simulink model "DCMotor"  (R2024b)
settings: Solver=VariableStepAuto  StartTime=0.0  StopTime=0.2  RelTol=1e-3
values from neighbouring files (symbols this model uses):
  b = 0    [C01A_Parameters.m]    (also in param.m = 0.000180072449898)
  Cn = 0.22    [C01A_Parameters.m]    (also in param.m = 0)
  J = 0.352e-4    (= 3.52e-05)    [C01A_Parameters.m]    (also in param.m)
  Km = 0.11    [C01A_Parameters.m]    (also in param.m)
  L = 4.1e-3    (= 0.0041)    [C01A_Parameters.m]    (also in param.m)
  R = 3.2    [C01A_Parameters.m]    (also in param.m)
  RadToRpm = 60/(2*pi)    (= 9.54929658551)    [C01A_Parameters.m]    (also in param.m)
settings Model: Creator=student  LastModifiedBy=student

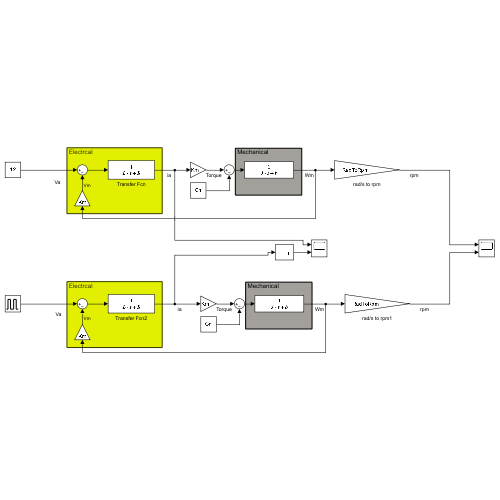
[thumbnail: Simulink's stored preview of the top-level diagram]
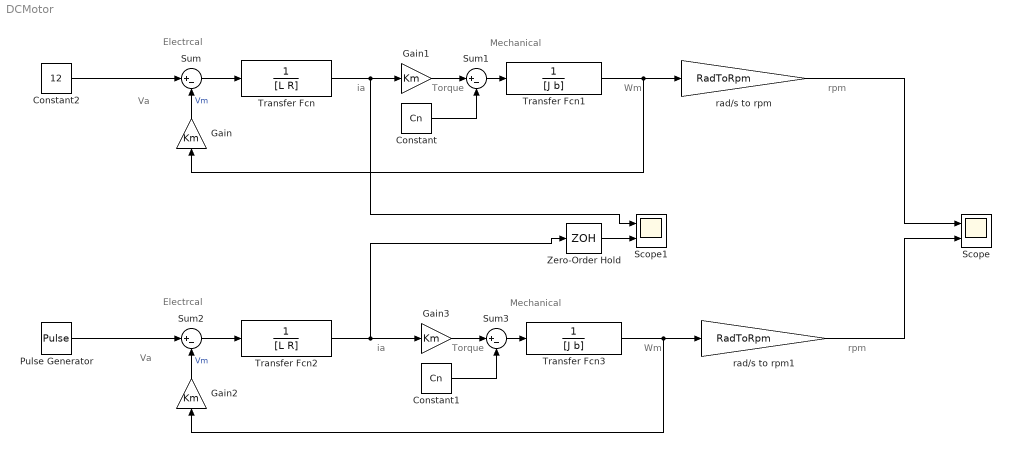
== system DCMotor ==
  note: Mechanical
  note: Electrcal
  note: Va
  note: Torque
  note: ia
  note: Wm
  note: rpm
  note: Wm
  note: Torque
  note: Electrcal
  note: Mechanical
  note: Va
  note: ia
  note: rpm
  Constant : Constant  Value=Cn
  Constant1 : Constant  Value=Cn
  Constant2 : Constant  Value=12
  Gain{,1..3} (4 alike) : Gain  Gain=Km
  Pulse Generator : DiscretePulseGenerator  PulseType=Time based  Amplitude=24  Period=0.001  PulseWidth=50
  Scope : Scope  NumInputPorts=2
  Scope1 : Scope  NumInputPorts=2
  Sum{,1..3} (4 alike) : Sum  Inputs=|+-
  Transfer Fcn : TransferFcn  Denominator=[L R]
  Transfer Fcn1 : TransferFcn  Denominator=[J b]
  Transfer Fcn2 : TransferFcn  Denominator=[L R]
  Transfer Fcn3 : TransferFcn  Denominator=[J b]
  Zero-Order Hold : ZeroOrderHold  SampleTime=-1
  rad/s to rpm : Gain  Gain=RadToRpm
  rad/s to rpm1 : Gain  Gain=RadToRpm
  wires:
  Constant2/1 -> Sum/1
  Gain/1 -> Sum/2  "Vm"
  Sum/1 -> Transfer Fcn/1
  Transfer Fcn/1 -> Scope1/1, Gain1/1
  Transfer Fcn1/1 -> Gain/1, rad/s to rpm/1
  Gain1/1 -> Sum1/1
  rad/s to rpm/1 -> Scope/1
  Sum1/1 -> Transfer Fcn1/1
  Constant/1 -> Sum1/2
  Constant1/1 -> Sum3/2
  Sum3/1 -> Transfer Fcn3/1
  Transfer Fcn3/1 -> Gain2/1, rad/s to rpm1/1
  Sum2/1 -> Transfer Fcn2/1
  Pulse Generator/1 -> Sum2/1
  Transfer Fcn2/1 -> Gain3/1, Zero-Order Hold/1
  Gain3/1 -> Sum3/1
  rad/s to rpm1/1 -> Scope/2
  Gain2/1 -> Sum2/2  "Vm"
  Zero-Order Hold/1 -> Scope1/2
